simulink model "ECU1119_18b_st"  (R2018b)
settings: Solver=FixedStepDiscrete  StartTime=0.0  StopTime=10.0  RelTol=1e-3
InitFcn:
  | mbd_mpc_consistency_checks(bdroot(gcs));
values from neighbouring files (symbols this model uses):
  ANRtarget = 1.05    [Engine_init.m]
  EGRKi = 0.03    [Engine_init.m]
  EGRKp = 1.2*3    (= 3.6)    [Engine_init.m]
  EGRMax = 1    [Engine_init.m]
  EGRMin = 0    [Engine_init.m]
  EGRTgt = [0.25,0.22,0.20,0.18,0.16,0.12,0.10 ... (first row only)    [Engine_init.m]
  EGRTgt_x = [700,1200,1400,1600,1800,2000,2200]    [Engine_init.m]
  EGRTgt_y = [20,60,100,140,160]    [Engine_init.m]
  EngineSpdTgt = [700:150:2200]    [Engine_init.m]
  EngineSpdTgt_x = [0:10:100]    [Engine_init.m]
  FuelCyleMax = [40,50,60,60,60 ... (first row only)    [Engine_init.m]
  FuelCyleMax_x = [120,180,240,300,360]    [Engine_init.m]
  FuelCyleMax_y = [700,1200,1400,1600,1800,2000,2200]    [Engine_init.m]
  FuelCyleMaxSw = 0    [Engine_init.m]
  FuelCyleMin = 10    [Engine_init.m]
  FuelKd = 0    [Engine_init.m]
  FuelKi = 0.009*5    (= 0.045)    [Engine_init.m]
  FuelKp = 0.03*5    (= 0.15)    [Engine_init.m]
  Regen_Enable_SW = true    [Engine_init.m]
  Soot_Load_Off = 4    [Engine_init.m]
  Soot_Load_On = 18    [Engine_init.m]
  T_regen_max = 680    [Engine_init.m]
  T_regen_min = 550    [Engine_init.m]
undefined symbols (not defined in the file or in its folder): fifo_0_vect, fifo_1_vect, LQFP, pts1_fifo_0_vect, pts1_fifo_1_vect, pts2_fifo_0_vect, pts2_fifo_1_vect, pts3_fifo_0_vect, pts3_fifo_1_vect, pts4_fifo_0_vect, pts4_fifo_1_vect
libraries: mbd_mpc574x_ec_toolbox x111, simulink x12, canmsglib x8
(part 5 of 5)

== system ECU1119_18b_st/SigIn/PWM/PWM_PTS3/Subsystem_capture ==
  In1 : Inport
  function : TriggerPort  TriggerType=function-call  VariantControl=Variant
  Constant : Constant  Value=0  OutDataTypeStr=uint8
  Counter Limited : simulink/Sources/Counter Limited  uplimit=255  tsamp=-1
  Data Store Write : DataStoreWrite  DataStoreName=pts3_pwm_cnt
  Data Store Write4 : DataStoreWrite  DataStoreName=pwm4_cnt
  Terminator : Terminator
  eTimer_Arm_Capture : mbd_mpc574x_ec_toolbox/Motor Control Blocks/eTIMER Blocks/eTimer_Arm_Capture  etimerModule=1  etimerChannel=1  etimerArmAction=Stop
      settings: SourceProductName=NXP Model-Based Design Toolbox for MPC57xx MCUs
  eTimer_Capture : mbd_mpc574x_ec_toolbox/Motor Control Blocks/eTIMER Blocks/eTimer_Capture  etimerModule=1  etimerChannel=1
      settings: SourceProductName=NXP Model-Based Design Toolbox for MPC57xx MCUs
  Out1 : Outport  OutDataTypeStr=uint16
  Out2 : Outport  Port=2  OutDataTypeStr=uint16
  Out3 : Outport  Port=3  OutDataTypeStr=uint16
  Out4 : Outport  Port=4  OutDataTypeStr=uint16
  wires:
  eTimer_Capture/1 -> Out1/1
  eTimer_Capture/4 -> Out4/1
  eTimer_Capture/3 -> Out3/1
  eTimer_Capture/2 -> Out2/1
  In1/1 -> Terminator/1
  Constant/1 -> Data Store Write/1
  Counter Limited/1 -> Data Store Write4/1

== system ECU1119_18b_st/SigIn/PWM/PWM_PTS4/Subsystem ==
  In1 : Inport
  Add2 : Sum  AccumDataTypeStr=single
  Constant : Constant  OutDataTypeStr=uint8
  Constant1 : Constant  Value=0  OutDataTypeStr=single
  Data Store Read3 : DataStoreRead  DataStoreName=pts4_pwm_cnt
  Data Store Write : DataStoreWrite  DataStoreName=pts4_pwm_cnt
  Saturation : Saturate  UpperLimit=100  LowerLimit=0
  Switch : Switch  Criteria=u2 > Threshold  Threshold=100
  Out1 : Outport  VectorParamsAs1DForOutWhenUnconnected=on
  wires:
  In1/1 -> Switch/3
  Constant/1 -> Add2/1
  Switch/1 -> Out1/1
  Constant1/1 -> Switch/1
  Data Store Read3/1 -> Add2/2
  Add2/1 -> Saturation/1, Switch/2
  Saturation/1 -> Data Store Write/1

== system ECU1119_18b_st/SigIn/PWM/PWM_PTS4/Subsystem_capture ==
  In1 : Inport
  function : TriggerPort  TriggerType=function-call  VariantControl=Variant
  Constant : Constant  Value=0  OutDataTypeStr=uint8
  Counter Limited : simulink/Sources/Counter Limited  uplimit=255  tsamp=-1
  Data Store Write : DataStoreWrite  DataStoreName=pts4_pwm_cnt
  Data Store Write1 : DataStoreWrite  DataStoreName=pwm1_cnt
  Terminator : Terminator
  eTimer_Arm_Capture : mbd_mpc574x_ec_toolbox/Motor Control Blocks/eTIMER Blocks/eTimer_Arm_Capture  etimerModule=0  etimerChannel=2  etimerArmAction=Stop
      settings: SourceProductName=NXP Model-Based Design Toolbox for MPC57xx MCUs
  eTimer_Capture : mbd_mpc574x_ec_toolbox/Motor Control Blocks/eTIMER Blocks/eTimer_Capture  etimerModule=0  etimerChannel=2
      settings: SourceProductName=NXP Model-Based Design Toolbox for MPC57xx MCUs
  Out1 : Outport  OutDataTypeStr=uint16
  Out2 : Outport  Port=2  OutDataTypeStr=uint16
  Out3 : Outport  Port=3  OutDataTypeStr=uint16
  Out4 : Outport  Port=4  OutDataTypeStr=uint16
  wires:
  Constant/1 -> Data Store Write/1
  In1/1 -> Terminator/1
  eTimer_Capture/2 -> Out2/1
  eTimer_Capture/3 -> Out3/1
  eTimer_Capture/4 -> Out4/1
  eTimer_Capture/1 -> Out1/1
  Counter Limited/1 -> Data Store Write1/1

== system ECU1119_18b_st/SigIn/PWM/Subsystem/Frequency_DutyCycle_Computation ==
  Add : Sum  Inputs=+-  AccumDataTypeStr=single
  Add1 : Sum  Inputs=+-  AccumDataTypeStr=single
  Data Store Read : DataStoreRead  DataStoreName=fifo_0_vect  DataStoreElements=fifo_0_vect(2)#fifo_0_vect(1)
  Data Store Read1 : DataStoreRead  DataStoreName=fifo_1_vect  DataStoreElements=fifo_1_vect(1)
  Data Store Read2 : DataStoreRead  DataStoreName=fifo_0_vect  DataStoreElements=fifo_0_vect(1)
  Divide : Product  Inputs=*/  OutDataTypeStr=single
  Divide1 : Product  Inputs=*//
  Freq_MC : Constant  Value=80000000  OutDataTypeStr=single
  Prescaler : Constant  Value=32  OutDataTypeStr=single
  Out1 : Outport
  Out2 : Outport  Port=2
  wires:
  Data Store Read1/1 -> Add1/1
  Data Store Read/2 -> Add/2
  Divide1/1 -> Out2/1
  Add/1 -> Divide/2, Divide1/3
  Add1/1 -> Divide/1
  Divide/1 -> Out1/1
  Data Store Read/1 -> Add/1
  Freq_MC/1 -> Divide1/1
  Prescaler/1 -> Divide1/2
  Data Store Read2/1 -> Add1/2

== system ECU1119_18b_st/SigIn/PWM/Subsystem/eTimer Configuration and Signal Measurements ==
  Subsystem_capture : Subsystem
  eTimer_Arm_Capture : mbd_mpc574x_ec_toolbox/Motor Control Blocks/eTIMER Blocks/eTimer_Arm_Capture  etimerModule=0  etimerChannel=1  etimerArmAction=Start
      settings: SourceProductName=NXP Model-Based Design Toolbox for MPC57xx MCUs
  eTimer_Config : mbd_mpc574x_ec_toolbox/Motor Control Blocks/eTIMER Blocks/eTimer_Config  etimerModule=0  etimerChannel=1  etimerMode=COUNT Mode  etimerCountOnce=Count repeatedly  etimerCountLength=Continue counting to roll over  etimerCountDirection=Count up  etimerCountStart=on  etimerCaptureArm=on  etimerShowAdv=on  etimerPrimarySource=IP Bus clock divide by 32 prescaler  etimerPrimaryPolarity=True polarity  etimerSecondarySource=Counter 0 input pin  etimerSecondaryPolarity=True polarity  etimerSampleCount=Require 3 consecutive samples to be of equal value  etimerSamplePeriod=0  etimerOutEnable=The external pin is configured as an input  etimerOutPolarity=True polarity  etimerOutMode=Toggle OFLAG output using alternating compare registers  etimerCompMode="COMP1 and COMP2  are used when the counter is counting up"  etimerCompLoad1=COMP1 is never preload  etimerCompLoad2=COMP2 is never preload  etimerCapt1=Capture rising edges  etimerCapt2=Capture falling edges  etimerOneShot=Free running mode is selected  etimerMasterMode=Disable broadcast of this channel output  etimerCoForce=Other channels cannot force this channel output  etimerCoChanInit=Other channels cannot force re-initialization of this channel  etimerRedundant=off  etimerCOMP1init=0  etimerCOMP2init=0  etimerCNTRinit=0  etimerCh0=PTA0: [eTimer0_ETC0 | eTimer_0 Input Data Channel 0]  etimerCh1=None  etimerCh2=None  etimerCh3=None  etimerCh4=None  etimerCh5=None  etimerIsrTCFIE=off  etimerIsrTCF1IE=off  etimerIsrTCF2IE=off  etimerIsrTOFIE=off  etimerIsrIELFIE=off  etimerIsrIEHFIE=off  etimerIsrICF1IE=off  etimerIsrICF2IE=on  etimerIsrRCF=off  etimerIsrWDF=off
      settings: SourceProductName=NXP Model-Based Design Toolbox for MPC57xx MCUs
  eTimer_ISR : mbd_mpc574x_ec_toolbox/Motor Control Blocks/eTIMER Blocks/eTimer_ISR_Handler  etimerModule=0  etimerInterrupt=Channel Interrupt  etimerChannel=1  etimerIsrPriority=14
      settings: SourceProductName=NXP Model-Based Design Toolbox for MPC57xx MCUs
  Out1 : Outport
  Out2 : Outport  Port=2
  Out3 : Outport  Port=3
  Out4 : Outport  Port=4
  wires:
  eTimer_ISR/1 -> Subsystem_capture/Trigger
  eTimer_ISR/2 -> Subsystem_capture/1(In1)
  Subsystem_capture/1(Out1) -> Out1/1
  Subsystem_capture/2(Out2) -> Out2/1
  Subsystem_capture/3(Out3) -> Out3/1
  Subsystem_capture/4(Out4) -> Out4/1

== system ECU1119_18b_st/SigIn/PWM/Subsystem/eTimer Configuration and Signal Measurements/Subsystem_capture ==
  In1 : Inport
  function : TriggerPort  TriggerType=function-call  VariantControl=Variant
  Terminator : Terminator
  eTimer_Arm_Capture : mbd_mpc574x_ec_toolbox/Motor Control Blocks/eTIMER Blocks/eTimer_Arm_Capture  etimerModule=0  etimerChannel=1  etimerArmAction=Stop
      settings: SourceProductName=NXP Model-Based Design Toolbox for MPC57xx MCUs
  eTimer_Capture : mbd_mpc574x_ec_toolbox/Motor Control Blocks/eTIMER Blocks/eTimer_Capture  etimerModule=0  etimerChannel=1
      settings: SourceProductName=NXP Model-Based Design Toolbox for MPC57xx MCUs
  Out1 : Outport  OutDataTypeStr=uint16
  Out2 : Outport  Port=2  OutDataTypeStr=uint16
  Out3 : Outport  Port=3  OutDataTypeStr=uint16
  Out4 : Outport  Port=4  OutDataTypeStr=uint16
  wires:
  eTimer_Capture/1 -> Out1/1
  eTimer_Capture/4 -> Out4/1
  eTimer_Capture/3 -> Out3/1
  eTimer_Capture/2 -> Out2/1
  In1/1 -> Terminator/1

== stateflow chart ECU1119_18b_st/ECU/ECU/DPF_REGEN/Chart ==
  state Idle
    en:Regen_Request=false; PostInj_Request=false;
    Regen_State = uint8(0);
  state Wait
    en,du:Regen_Request=true;
    PostInj_Request =(ExhTemp_DPF_in_c < T_regen_min);
    Regen_State = uint8(1);
  state Regen
    en,du: Regen_Request=true;
    Regen_State = uint8(2);
  (default) -> Idle
  Idle -> Wait : [DPF_SootLoad > Soot_Load_On && Regen_Enable_SW==true]
  Regen -> Idle [order 1] : [(ExhTemp_DPF_in_c > T_regen_max)||(DPF_SootLoad < Soot_Load_Off)]
  Wait -> Regen : [ExhTemp_DPF_in_c > T_regen_min]
  Regen -> Wait [order 2] : [ExhTemp_DPF_in_c <0.9*T_regen_min]
  data: DPF_SootLoad input; ExhTemp_DPF_in_c input; Regen_Request output boolean; Regen_State output uint8; PostInj_Request output boolean; T_regen_min parameter; T_regen_max parameter; Soot_Load_On parameter; Soot_Load_Off parameter; Regen_Enable_SW parameter

== stateflow chart ECU1119_18b_st/Init/Init/Chart ==
  state POWER_ON
    LS001 = 1;
  state POWER_HOLD
    LS001 = 1;
  state POWER_OFF
    LS001 = 0;
  (default) -> POWER_ON
  POWER_HOLD -> POWER_ON [order 1] : [KeyOn==1]
  POWER_ON -> POWER_HOLD : [KeyOn==0]
  POWER_HOLD -> POWER_OFF [order 2] : [after(5,sec)]
  data: LS001 output; KeyOn input

== stateflow chart ECU1119_18b_st/GPIO /PWM_OUT/FreqCMD ==
  settings: executeAtInitialization=1
  state A
    du:
    freq = 20000;
    cntr = cntr + 1;
    dc = 0.25;
  state A1
    du:
    freq = 10000;
    cntr = cntr - 1;
    dc =  0.5;
  (default) -> A : {cntr=0;dc=0;}
  A1 -> A : [cntr < 1]
  A -> A1 : [cntr > 50]
  data: cntr local uint32 =0; freq output uint32; dc output single

== stateflow chart ECU1119_18b_st/Initialization & SPI timer1/CS1 LS/Chart ==
  state clear
    en:high=128+7;low=1;cnt=0;
    du:cnt = cnt + 1;
  state en
    en:high=128+1+64;low=0;cnt=0;
    du:cnt = cnt + 1;
  state config
    en:high=128+7+64;low=1+128;cnt=0;
    du:cnt = cnt + 1;
  (default) -> clear
  clear -> en : [cnt>5]
  en -> config : [cnt>5]
  data: high output; low output; cnt local

== stateflow chart ECU1119_18b_st/Initialization & SPI timer1/CS3 LS/Chart ==
  state ConfigA
    en:high=80+mode*(1+4);low=0+mode*(1+4);cnt=0;
    du:cnt = cnt + 1;
  state en
    en:high=96;low=0;cnt=0;
  (default) -> ConfigA
  ConfigA -> en : [cnt>4]
  data: high output; low output; cnt local; mode input

== stateflow chart ECU1119_18b_st/Initialization & SPI timer1/CS5 LS/Chart ==
  state clear
    en:high=128+7;low=1;cnt=0;
    du:cnt = cnt + 1;
  state en
    en:high=128+1+64;low=0;cnt=0;
    du:cnt = cnt + 1;
  state config
    en:high=128+7+64;low=1+128;cnt=0;
  (default) -> clear
  clear -> en : [cnt>5]
  en -> config : [cnt>5]
  data: high output; low output; cnt local

== stateflow chart ECU1119_18b_st/Initialization & SPI timer1/Chart ==
  state Idle
    en:Flg=0;
  state Initialize
    en:Flg=1;
  state Normal
    en:Flg=2;
  (default) -> Idle
  Normal -> Idle : [ResetFlg==1]
  Initialize -> Idle [order 2] : [ResetFlg==1]
  Idle -> Initialize : [ResetFlg==0]
  Initialize -> Normal [order 1] : [InitFlg>0]
  data: ResetFlg input; InitFlg input; Flg output

== stateflow chart ECU1119_18b_st/Initialization & SPI timer1/Chart1 ==
  state IDLE
    en:Flg=0;
  state CS1
    en:Flg=1;cnt=0;
    du:cnt = cnt + 1;
  state CS5
    en:Flg=2;cnt=0;
    du:cnt = cnt + 1;
  state Done
    en:Flg=9;
  (default) -> IDLE
  Done -> IDLE : [VcuMode==0]
  IDLE -> CS1 : [VcuMode==1]
  CS1 -> CS5 : [cnt>20]
  CS5 -> Done : [cnt>20]
  data: VcuMode input; Flg output; cnt local

== stateflow chart ECU1119_18b_st/Initialization & SPI timer1/Chart2 ==
  state IDLE
    en:Flg=0;
  state CS2
    en:Flg=1;cnt=0;
    du:cnt = cnt + 1;
  state CS3
    en:Flg=2;cnt=0;
    du:cnt = cnt + 1;
  state Done
    en:Flg=9;
  (default) -> IDLE
  Done -> IDLE : [VcuMode==0]
  IDLE -> CS2 : [VcuMode==1]
  CS2 -> CS3 : [cnt>20]
  CS3 -> Done : [cnt>20]
  data: VcuMode input; Flg output; cnt local
